simulink model "HVAC_Thermal_Plant_Discrete"  (R2022b)
settings: Solver=FixedStepDiscrete  StartTime=0  StopTime=100  FixedStep=0.1  RelTol=1e-3
settings Model: Creator=Utilisateur  LastModifiedBy=Utilisateur
settings OptimizationCC: UseDivisionForNetSlopeComputation=on
settings ModelReferenceCC: ModelReferenceMinAlgLoopOccurrences=on

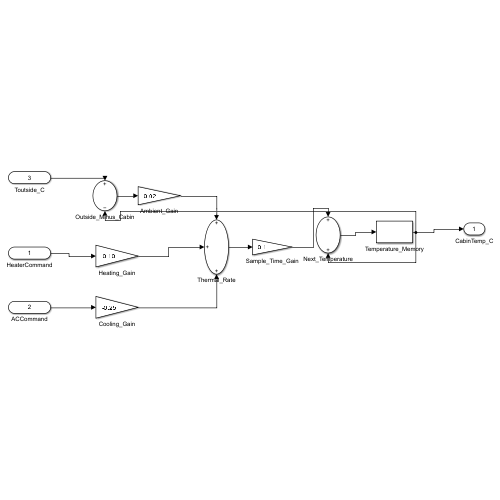
[thumbnail: Simulink's stored preview of the top-level diagram]
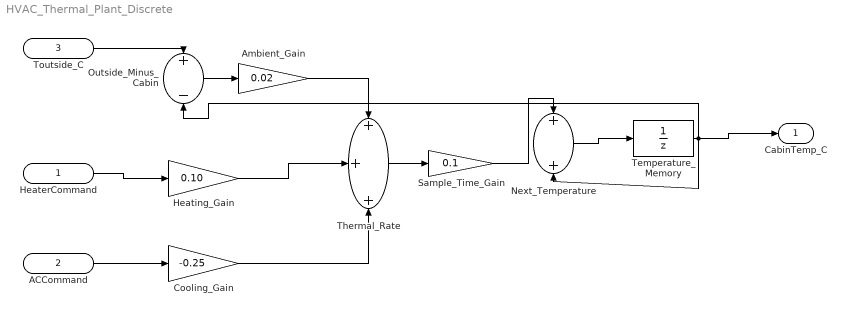
== system HVAC_Thermal_Plant_Discrete ==
  HeaterCommand : Inport
  ACCommand : Inport  Port=2
  Toutside_C : Inport  Port=3
  Ambient_Gain : Gain  Gain=0.02
  Cooling_Gain : Gain  Gain=-0.25
  Heating_Gain : Gain  Gain=0.10
  Next_Temperature : Sum
  Outside_Minus_Cabin : Sum  Inputs=+-
  Sample_Time_Gain : Gain  Gain=0.1
  Temperature_Memory : UnitDelay  InitialCondition=18  SampleTime=0.1  HasFrameUpgradeWarning=on
  Thermal_Rate : Sum  Inputs=+++
  CabinTemp_C : Outport
  wires:
  Toutside_C/1 -> Outside_Minus_Cabin/1
  Temperature_Memory/1 -> Outside_Minus_Cabin/2, Next_Temperature/2, CabinTemp_C/1
  Outside_Minus_Cabin/1 -> Ambient_Gain/1
  HeaterCommand/1 -> Heating_Gain/1
  ACCommand/1 -> Cooling_Gain/1
  Ambient_Gain/1 -> Thermal_Rate/1
  Heating_Gain/1 -> Thermal_Rate/2
  Cooling_Gain/1 -> Thermal_Rate/3
  Thermal_Rate/1 -> Sample_Time_Gain/1
  Sample_Time_Gain/1 -> Next_Temperature/1
  Next_Temperature/1 -> Temperature_Memory/1
